simulink model "ssc_hydromech_power_split_cvt"  (R2025a)
settings: Solver=VariableStepAuto  StartTime=0.0  StopTime=200  RelTol=1e-3
StartFcn:
  | tic
StopFcn:
  | Elapsed_Sim_Time = toc;
  | disp(['Elapsed Sim Time = ' num2str(Elapsed_Sim_Time)]);
undefined symbols (not defined in the file or in its folder): HMPST
libraries: sm_wheel_loader_lib x8, fl_lib x7, sdl_lib x2, simulink x1, nesl_utility x1
Description:
  | Hydromechanical Power Split CVT
  | Copyright 2023-2025 The MathWorks, Inc.
settings Model: PacingRate=10  TunableVars=Init_Veh_TopSpeed  TunableVarsStorageClass=Auto  Creator=Shusen Zhang  LastModifiedBy=smiller
settings SolverCC: MaxConsecutiveMinStep=5
settings DataIOCC: ReturnWorkspaceOutputs=off  SignalLoggingName=logsout_ssc_hydromech_power_split_cvt
settings DebuggingCC: UnderspecifiedInitializationDetection=Classic  MergeDetectMultiDrivingBlocksExec=none
settings ModelReferenceCC: PropagateSignalLabelsOutOfModel=off
settings RTWCC: GPUComputeCapability=3.5
settings SimscapeCC: SimscapeLogType=all  SimscapeLogName=simlog_ssc_hydromech_power_split_cvt  SimscapeLogLimitData=off
settings ExplorerConfigSet: SimMechanicsOpenEditorOnUpdate=off

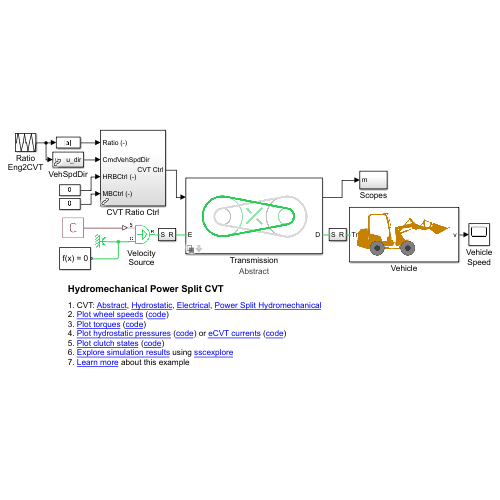
[thumbnail: Simulink's stored preview of the top-level diagram]
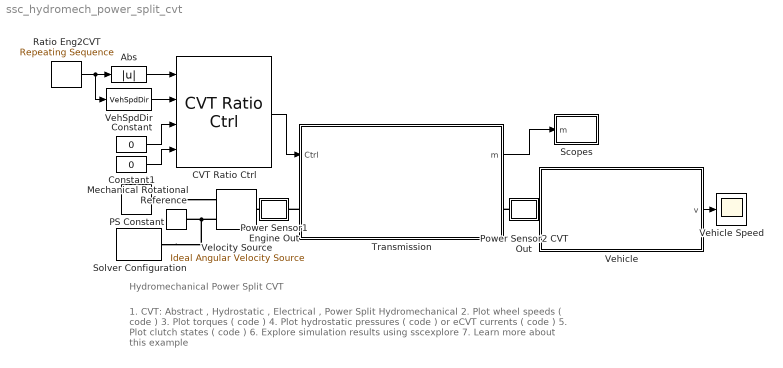
== system ssc_hydromech_power_split_cvt ==
  note: Hydromechanical Power Split CVT
  note: 1. CVT: Abstract , Hydrostatic , Electrical , Power Split Hydromechanical
      | 2. Plot wheel speeds ( code )
      | 3. Plot torques ( code )
      | 4. Plot hydrostatic pressures ( code ) or eCVT currents ( code )
      | 5. Plot clutch states ( code )
      | 6. Explore simulation results using sscexplore
      | 7. Learn more about this example
  Abs : Abs  ZeroCross=off  SaturateOnIntegerOverflow=off
  CVT Ratio Ctrl : sm_wheel_loader_lib/Controller/CVT Ratio Ctrl  SystemSampleTime=-1  VariantActivationTime=update diagram  EmptyChoice=off  PassThrough=off  PassThroughVariantControl=(default)  EmptyChoiceVariantControl=(default)  AllowFlexibleInterface=on  Latency=0  AutoFrameSizeCalculation=off
  Constant : Constant  Value=0
  Constant1 : Constant  Value=0
  Mechanical Rotational Reference : fl_lib/Mechanical/Rotational Elements/Mechanical Rotational Reference
  PS Constant : fl_lib/Physical Signals/Sources/PS Constant  constant=2200 rpm
  Power Sensor1 Engine Out : Subsystem
  Power Sensor2 CVT Out : Subsystem
  Ratio Eng2CVT : simulink/Sources/Repeating Sequence  rep_seq_t=[0 5 95 105 195 200 205 295 305 395 400]/2  rep_seq_y=[0 0 2.1 2.1 0 0 0 -2.1 -2.1 0 0]
  Scopes : Subsystem
  Solver Configuration : nesl_utility/Solver Configuration  PhysicalDomain=network_engine_domain  SubClassName=solver  LeftPortType=input  RightPortType=generic  Tones=[]  Harmonics=[]  SimulateNoise=off  Profile=off  UseLocalSampling=off  EnableSwitchedLinearOptims=on  FrequencyDomain=off  UseCCode=off  RelTol=0.001  AbsTol=1e-06  MinStep=1e-09  ToWorkspace=off  RevertToSquareIcSolve=off  NumHomotopyIterations=100  PhasorMode=off  PhasorModeNumHarmonics=1  ConsistencySolver=NEWTON_XTOL_AFTER_FTOL  IndexReductionMethod=DerivativeReplacement  DoDC=off  ResidualTolerance=1e-09  ConsistencyTolSource=GLOBAL  ConsistencyAbsTol=0.001  ConsistencyRelTol=0.001  ConsistencyTolFactor=0.001  UseLocalSolver=off  LocalSolverChoice=NE_BACKWARD_EULER_ADVANCER  ResolveIndetEquations=on  FunctionEvalNumThread=1  LocalSolverSampleTime=0.001  DoFixedCost=off  MaxNonlinIter=1  MaxModeIter=2  ComputeImpulses=off  ImpulseIterations=2  LinearAlgebra=Sparse  LinearAlgebraNumThread=0  EquationFormulation=NE_TIME_EF  DelaysMemoryBudget=1024  AutomaticFiltering=on  FilteringTimeConstant=0.001  PartitionStorageMethod=AS_NEEDED  PartitionMemoryBudget=1024  PartitionMethod=FAST  MultibodyUseLocalSolver=off  MultibodyLocalSolverChoice=ODE1  MultibodyLocalSolverSampleTime=0.001
  Transmission : Subsystem  Variant=on  VariantControlMode=label  VariantControl=Choice  LabelModeActiveChoice=Abstract
      settings: AttributesFormatString=%<LabelModeActiveChoice>
  VehSpdDir : sm_wheel_loader_lib/Controller/Desired Ratio Calc/VehSpdDir  SystemSampleTime=-1  VariantActivationTime=update diagram  EmptyChoice=off  PassThrough=off  PassThroughVariantControl=(default)  EmptyChoiceVariantControl=(default)  AllowFlexibleInterface=on  Latency=0  AutoFrameSizeCalculation=off
  Vehicle : Subsystem
      mask Display: image('sm_wheel_loader_vehicle1D_IMAGE.png');
  Vehicle Speed : Scope
      settings: ActiveDisplayYMinimum=-37.51249  ActiveDisplayYMaximum=37.51245
  Velocity Source : fl_lib/Mechanical/Mechanical Sources/Ideal Angular Velocity Source
  wires:
  Transmission/1(m) -> Scopes/1(m)
  CVT Ratio Ctrl/1 -> Transmission/1(Ctrl)
  Constant/1 -> CVT Ratio Ctrl/3
  Constant1/1 -> CVT Ratio Ctrl/4
  Vehicle/1(v) -> Vehicle Speed/1
  Ratio Eng2CVT/1 -> Abs/1, VehSpdDir/1
  VehSpdDir/1 -> CVT Ratio Ctrl/2
  Abs/1 -> CVT Ratio Ctrl/1
  connections:
  Transmission/LConn1 -- Power Sensor1 Engine Out/RConn1
  Velocity Source/RConn2 -- Solver Configuration/RConn1 -- Mechanical Rotational Reference/LConn1
  PS Constant/RConn1 -- Velocity Source/RConn1
  Power Sensor2 CVT Out/RConn1 -- Vehicle/LConn1
  Power Sensor1 Engine Out/LConn1 -- Velocity Source/LConn1
  Power Sensor2 CVT Out/LConn1 -- Transmission/RConn1

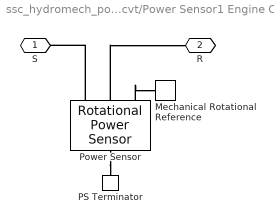
== system ssc_hydromech_power_split_cvt/Power Sensor1 Engine Out ==
  Mechanical Rotational Reference : fl_lib/Mechanical/Rotational Elements/Mechanical Rotational Reference
  PS Terminator : fl_lib/Physical Signals/Sinks/PS Terminator
  Power Sensor : sdl_lib/Sensors/Rotational Power Sensor  measurement_type=sdl.enum.rotationalPowerSensorType.instantaneous  averaging_period=1 s  max_frequency=1000 Hz  max_speed=1000 rpm
      settings: InternalSimscapePortConfiguration="{\"Bottom\":[],\"Left\":[{\"id\":\"S\",\"label\":\"S\",\"type\":\"foundation.mechanical.rotational.rotational\"},{\"id\":\"R\",\"label\":\"R\",\"type\":\"foundation.mechanical.rotational.rotational\"},{\"id\":\"C\",\"label\":\"C\",\"type\":\"foundation.mechanical.rotational.rotational\"}],\"Right\":[{\"id\":\"P\",\"label\":\"P\",\"type\":\"output\"}],\"Top\":[]}"
  S : PMIOPort  Side=Left
  R : PMIOPort  Port=2  Side=Right
  connections:
  Power Sensor/RConn1 -- PS Terminator/LConn1
  Power Sensor/LConn3 -- Mechanical Rotational Reference/LConn1
  Power Sensor/LConn2 -- R/RConn1
  Power Sensor/LConn1 -- S/RConn1

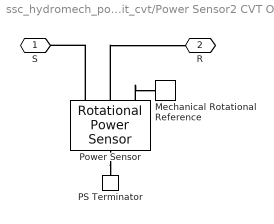
== system ssc_hydromech_power_split_cvt/Power Sensor2 CVT Out ==
  Mechanical Rotational Reference : fl_lib/Mechanical/Rotational Elements/Mechanical Rotational Reference
  PS Terminator : fl_lib/Physical Signals/Sinks/PS Terminator
  Power Sensor : sdl_lib/Sensors/Rotational Power Sensor  measurement_type=sdl.enum.rotationalPowerSensorType.instantaneous  averaging_period=1 s  max_frequency=1000 Hz  max_speed=1000 rpm
      settings: InternalSimscapePortConfiguration="{\"Bottom\":[],\"Left\":[{\"id\":\"S\",\"label\":\"S\",\"type\":\"foundation.mechanical.rotational.rotational\"},{\"id\":\"R\",\"label\":\"R\",\"type\":\"foundation.mechanical.rotational.rotational\"},{\"id\":\"C\",\"label\":\"C\",\"type\":\"foundation.mechanical.rotational.rotational\"}],\"Right\":[{\"id\":\"P\",\"label\":\"P\",\"type\":\"output\"}],\"Top\":[]}"
  S : PMIOPort  Side=Left
  R : PMIOPort  Port=2  Side=Right
  connections:
  Power Sensor/LConn1 -- S/RConn1
  Power Sensor/LConn2 -- R/RConn1
  Power Sensor/LConn3 -- Mechanical Rotational Reference/LConn1
  Power Sensor/RConn1 -- PS Terminator/LConn1

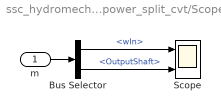
== system ssc_hydromech_power_split_cvt/Scopes ==
  m : Inport
  Bus Selector : BusSelector  OutputSignals=wIn,OutputShaft
  Scope : Scope  NumInputPorts=2
      settings: ActiveDisplayYMinimum=4647.37296  ActiveDisplayYMaximum=4651.03483  DataLoggingVariableName=ScopeData4
  wires:
  Bus Selector/2 -> Scope/2  "<OutputShaft>"
  Bus Selector/1 -> Scope/1  "<wIn>"
  m/1 -> Bus Selector/1

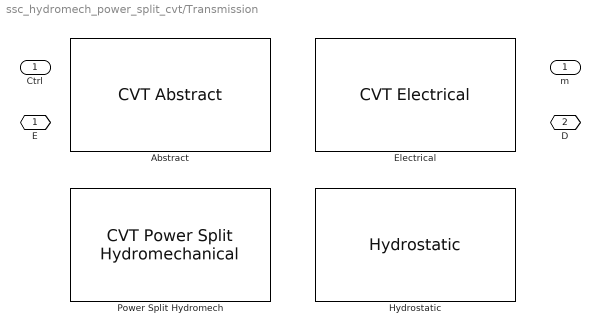
== system ssc_hydromech_power_split_cvt/Transmission ==
  Ctrl : Inport
  Abstract : sm_wheel_loader_lib/CVT Abstract  VariantControl=Abstract  dShaftE=HMPST.AbstractCVT.dInput  dShaftD=HMPST.AbstractCVT.dOutput  k=HMPST.AbstractCVT.kCompliance  d=HMPST.AbstractCVT.dCompliance
  Electrical : sm_wheel_loader_lib/CVT Electrical  VariantControl=Electrical
  Hydrostatic : sm_wheel_loader_lib/Hydrostatic  SystemSampleTime=-1  VariantControl=Hydrostatic  VariantActivationTime=update diagram  EmptyChoice=off  PassThrough=off  PassThroughVariantControl=(default)  EmptyChoiceVariantControl=(default)  AllowFlexibleInterface=on  Latency=0  AutoFrameSizeCalculation=off
  Power Split Hydromech : sm_wheel_loader_lib/CVT Power Split Hydromechanical  SystemSampleTime=-1  VariantControl=Power_Split_HM  VariantActivationTime=update diagram  EmptyChoice=off  PassThrough=off  PassThroughVariantControl=(default)  EmptyChoiceVariantControl=(default)  AllowFlexibleInterface=on  Latency=0  AutoFrameSizeCalculation=off
      settings: LibrarySourceBlock=sm_wheel_loader_lib/CVT Powersplit Hydromechanical
  E : PMIOPort  Side=Left
  D : PMIOPort  Port=2  Side=Right
  m : Outport

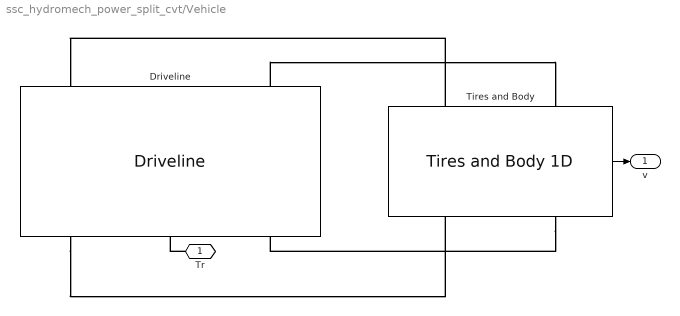
== system ssc_hydromech_power_split_cvt/Vehicle ==
  Driveline : sm_wheel_loader_lib/Wheel Loader Vehicle/Driveline/Driveline/Driveline 1D/Driveline  SystemSampleTime=-1  VariantActivationTime=update diagram  EmptyChoice=off  PassThrough=off  PassThroughVariantControl=(default)  EmptyChoiceVariantControl=(default)  AllowFlexibleInterface=on  Latency=0  AutoFrameSizeCalculation=off
  Tires and Body : sm_wheel_loader_lib/Tires and Body 1D  SystemSampleTime=-1  VariantActivationTime=update diagram  EmptyChoice=off  PassThrough=off  PassThroughVariantControl=(default)  EmptyChoiceVariantControl=(default)  AllowFlexibleInterface=on  Latency=0  AutoFrameSizeCalculation=off
      settings: PortSchema="{\"entries\":[{\"content\":{\"sides\":[{\"content\":{\"connectorIds\":[\"LConn1\",\"LConn2\"]},\"type\":\"ConnectorPlacement.EquallySpacedRectSide\",\"uuid\":\"f6e4eca3-fb02-4523-87a7-c8328825f67f\"},{\"content\":{\"connectorIds\":[\"RConn1\",\"RConn2\"],\"side\":\"RIGHT\"},\"type\":\"ConnectorPlacement.EquallySpacedRectSide\",\"uuid\":\"a01e7d42-3992-448e-add1-f2755d8f064c\"},{\"content\":{\"connectorIds\":[\"Out1\"],\"side\":\"TOP\"},\"type\":\"ConnectorPlacement.EquallySpacedRectSide\",\"uuid\":\"cf483cf6-51ef-4c82-b2ec-fd42745a5c51\"},{\"content\":{\"side\":\"BOTTOM\"},\"type\":\"ConnectorPlacement.EquallySpacedRectSide\",\"uuid\":\"9bbb772c-3b9f-4e30-8c40-373d820ff5eb\"}]},\"type\":\"ConnectorPlacement.EquallySpacedConnector\",\"uuid\":\"52398d34-f462-4e1c-abff-1dda3b221c82\"}],\"packageUris\":[\"http://schema.mathworks.com/mf0/Connector/R2020b\"],\"version\":\"1.0\"}"
  Tr : PMIOPort  Side=Left
  v : Outport
  wires:
  Tires and Body/1 -> v/1
  connections:
  Driveline/LConn3 -- Tires and Body/LConn1
  Tires and Body/LConn2 -- Driveline/LConn1
  Tires and Body/RConn1 -- Driveline/RConn3
  Driveline/RConn1 -- Tires and Body/RConn2
  Tr/RConn1 -- Driveline/RConn2
